simulink model "SwitchingLegTest"  (R2026b)
settings: Solver=FixedStepDiscrete  StopTime=fixtureCfg.Duration  FixedStep=experimentCfg.Step
PostLoadFcn:
  | addpath(fullfile(fileparts(fileparts(fileparts(fileparts(fileparts(get_param(bdroot,'FileName')))))),'docs','scripts'));initialize_motor_paths();initialize_motor_model(bdroot);
model workspace (MAT data in the model file):
  currentCfg.Ts = 0.0001
  currentCfg.BandwidthHz = 500
  currentCfg.Kpd = 3.14159265359
  currentCfg.Kpq = 3.76991118431
  currentCfg.Kid = 1570.79632679
  currentCfg.Kiq = 1570.79632679
  currentCfg.Kaw = 1000
  deadtimeCfg.DeadTime = 2e-06
  deadtimeCfg.DeviceDrop = 0
  deadtimeCfg.CurrentBlend = 0.1
  deadtimeCfg.ModelEnable = 0
  deadtimeCfg.CompensationEnable = 0
  deadtimeCfg.CompensationScale = 1
  deadtimeCfg.SwitchingStep = 1e-07
  experimentCfg.Step = 1e-07
  experimentCfg.LogTs = 1e-07
  experimentCfg.Duration = 1.5
  experimentCfg.Mode = 2
  experimentCfg.UseInverter = 1
  experimentCfg.UseTiming = 1
  experimentCfg.UseMechanical = 1
  experimentCfg.ImposedElectricalSpeed = 0
  experimentCfg.IdReference = 0
  experimentCfg.IqReference = 2
  experimentCfg.IqInitial = 0
  experimentCfg.SpeedReference = 40
  experimentCfg.SpeedInitial = 0
  experimentCfg.PositionReference = 1
  experimentCfg.PositionInitial = 0
  experimentCfg.CommandTime = 0.05
  experimentCfg.LoadTorque = 0.1
  experimentCfg.LoadTime = 0.35
  experimentCfg.Enable = 1
  experimentCfg.Reset = 0
  feedforwardCfg.Enable = 0
  feedforwardCfg.ParameterScale = 1
  fixtureCfg.Ts = 1e-07
  fixtureCfg.Duration = 0.001
  fixtureCfg.SolverStep = 1e-07
  fixtureCfg.Duty = 0.5
  fixtureCfg.Current = 3
  fixtureCfg.PwmPeriod = 0.0001
  fixtureCfg.Inputs = [1 1 1 1 1 1 1 1 1 1 1 1 ... (20002 elements, 10001x2)]
  inverterCfg.Vdc = 48
  inverterCfg.MinDuty = 0.02
  inverterCfg.PwmTs = 0.0001
  inverterCfg.LinearLimit = 26.6043004043
  motionCfg.Ts = 0.001
  motionCfg.NaturalFrequency = 20
  motionCfg.Damping = 0.9
  motionCfg.Kt = 0.21
  motionCfg.Kp = 0.0852380952381
  motionCfg.Ki = 0.952380952381
  motionCfg.Kaw = 20
  motionCfg.PositionKp = 8
  motionCfg.SpeedLimit = 80
  motionCfg.AccelerationLimit = 200
  motionCfg.CurrentLimit = 8
  pmsmCfg.Rs = 0.5
  pmsmCfg.Ld = 0.001
  pmsmCfg.Lq = 0.0012
  pmsmCfg.Flux = 0.035
  pmsmCfg.PolePairs = 4
  pmsmCfg.J = 0.0005
  pmsmCfg.B = 0.0001
  pmsmCfg.Id0 = 0
  pmsmCfg.Iq0 = 0
  pmsmCfg.Speed0 = 0
  pmsmCfg.Position0 = 0
  testStim.time = []
  testStim.signals.values = [1 1 1 1 1 1 1 1 1 1 1 1 ... (20002 elements, 10001x2)]
  testStim.signals.dimensions = 2
  timingCfg.Ts = 0.0001
  timingCfg.FeedbackTicks = 1
  timingCfg.ActuationTicks = 1
libraries: Deadtime x1
settings Model: Creator=24322  LastModifiedBy=24322

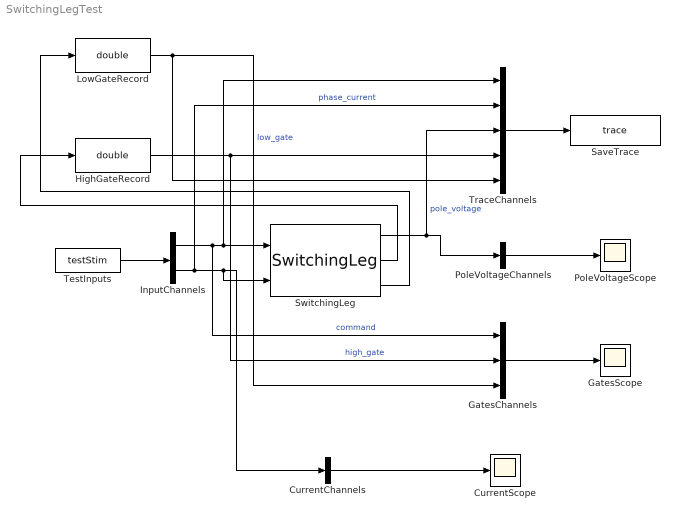
== system SwitchingLegTest ==
  CurrentChannels : Mux  Inputs=1
  CurrentScope : Scope
      settings: Title=Current  YLabel=A
  GatesChannels : Mux  Inputs=3
  GatesScope : Scope
      settings: Title=Gates  YLabel=1
  HighGateRecord : DataTypeConversion  OutDataTypeStr=double  SaturateOnIntegerOverflow=off  RndMeth=Floor
  InputChannels : Demux  Outputs=2
  LowGateRecord : DataTypeConversion  OutDataTypeStr=double  SaturateOnIntegerOverflow=off  RndMeth=Floor
  PoleVoltageChannels : Mux  Inputs=1
  PoleVoltageScope : Scope
      settings: Title=PoleVoltage  YLabel=V
  SaveTrace : ToWorkspace  VariableName=trace  SaveFormat=Structure With Time  SampleTime=experimentCfg.LogTs
  SwitchingLeg : Deadtime/SwitchingLeg  SystemSampleTime=-1  VariantActivationTime=update diagram  EmptyChoice=off  PassThrough=off  PassThroughVariantControl=(default)  EmptyChoiceVariantControl=(default)  AllowFlexibleInterface=on  Latency=0  AutoFrameSizeCalculation=off
  TestInputs : FromWorkspace  VariableName=testStim  SampleTime=deadtimeCfg.SwitchingStep  Interpolate=off  OutputAfterFinalValue=Holding final value
  TraceChannels : Mux  Inputs=5
  wires:
  CurrentChannels/1 -> CurrentScope/1
  PoleVoltageChannels/1 -> PoleVoltageScope/1
  GatesChannels/1 -> GatesScope/1
  SwitchingLeg/1 -> TraceChannels/3, PoleVoltageChannels/1  "pole_voltage"
  TraceChannels/1 -> SaveTrace/1
  InputChannels/2 -> SwitchingLeg/2, CurrentChannels/1, TraceChannels/2  "phase_current"
  InputChannels/1 -> SwitchingLeg/1, TraceChannels/1, GatesChannels/1  "command"
  TestInputs/1 -> InputChannels/1
  LowGateRecord/1 -> GatesChannels/3, TraceChannels/5  "low_gate"
  HighGateRecord/1 -> GatesChannels/2, TraceChannels/4  "high_gate"
  SwitchingLeg/2 -> HighGateRecord/1
  SwitchingLeg/3 -> LowGateRecord/1
